simulink model "aero2_position_integral_R2021a"  (R2021a)
settings: Solver=ode1  StartTime=0.0  StopTime=60  FixedStep=0.002  RelTol=1e-3
model workspace (MAT data in the model file):
  Dpos = 5.83392170192
  Dq = 3.88928113461
  Kaw = 20
  Kff = 1
  Ki = 1.84164606325
  Kint = 7.35390515018
  Kp = 0.216370391856
  Kpos = 11.344880808
  Kq = 3.78162693601
  Kref = 3.78162693601
  ReferenceRate = [0 0.002 0.004 0.006 0.008 0.01 0.012 0.014 0.016 0.018 0.02 0.022 ... (90003 elements, 30001x3)]
  U_h : timeseries (value not decoded)
  U_v : timeseries (value not decoded)
  X0 = [0; 0; 0; 0]
  meas_on = 0
(part 2 of 2)

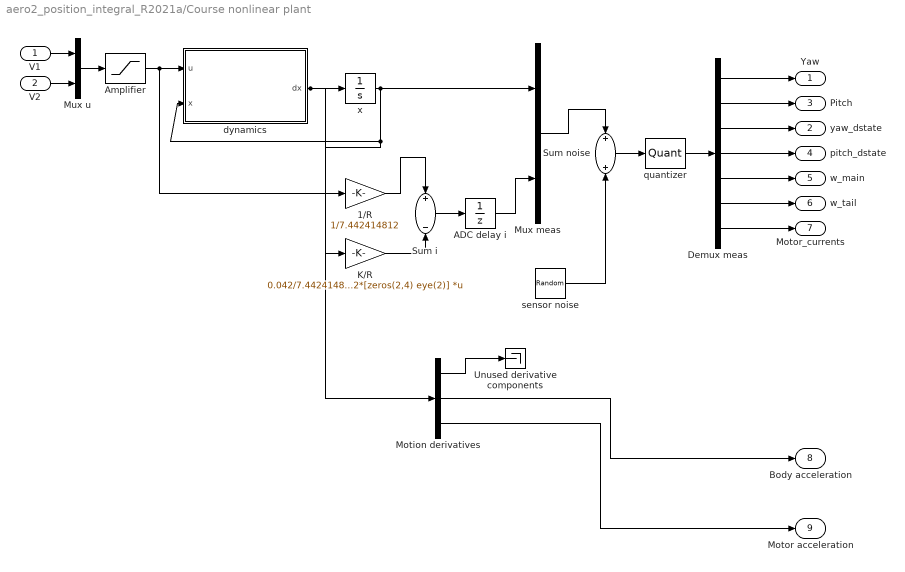
== system aero2_position_integral_R2021a/Course nonlinear plant ==
  V1 : Inport
  V2 : Inport  Port=2
  1/R : Gain  Gain=1/7.442414812
  ADC delay i : UnitDelay  InitialCondition=[0;0]  SampleTime=0.002
  Amplifier : Saturate  UpperLimit=24  LowerLimit=-24
  Demux meas : Demux  Outputs=[1 1 1 1 1 1 2]
  K/R : Gain  Gain=0.042/7.442414812*[zeros(2,4) eye(2)]  Multiplication=Matrix(K*u)
  Motion derivatives : Demux  Outputs=[2 2 2]
  Mux meas : Mux  Inputs=[6 2]
  Mux u : Mux  Inputs=2
  Sum i : Sum  Inputs=+-
  Sum noise : Sum
  Unused derivative components : Terminator
  dynamics : MATLAB Function  TreatAsAtomicUnit=on
  quantizer : Quantizer  QuantizationInterval=max((meas)*[0.0015339807878856412;0.0030679615757712823;0.001;0.001;0.050000000000000003;0.050000000000000003;0.001;0.001], 1e-12)
  sensor noise : RandomNumber  Mean=zeros(8,1)  Variance=((meas)*[0.0005;0.0005;0.005;0.005;0.3;0.3;0.01;0.01]).^2  Seed=[61027;18839;4421;30893;23341;7781;51117;9013]  SampleTime=0.002
  x : Integrator  InitialCondition=zeros(6,1)
  Yaw : Outport
  yaw_dstate : Outport  Port=2
  Pitch : Outport  Port=3
  pitch_dstate : Outport  Port=4
  w_main : Outport  Port=5
  w_tail : Outport  Port=6
  Motor_currents : Outport  Port=7
  Body acceleration : Outport  Port=8
  Motor acceleration : Outport  Port=9
  wires:
  Demux meas/7 -> Motor_currents/1
  Demux meas/6 -> w_tail/1
  Demux meas/5 -> w_main/1
  Demux meas/4 -> pitch_dstate/1
  Demux meas/2 -> Pitch/1
  Demux meas/3 -> yaw_dstate/1
  Demux meas/1 -> Yaw/1
  quantizer/1 -> Demux meas/1
  Sum noise/1 -> quantizer/1
  sensor noise/1 -> Sum noise/2
  Mux meas/1 -> Sum noise/1
  ADC delay i/1 -> Mux meas/2
  Sum i/1 -> ADC delay i/1
  K/R/1 -> Sum i/2
  1/R/1 -> Sum i/1
  x/1 -> K/R/1, dynamics/2(x), Mux meas/1
  dynamics/1(dx) -> x/1, Motion derivatives/1
  Amplifier/1 -> 1/R/1, dynamics/1(u)
  Mux u/1 -> Amplifier/1
  V2/1 -> Mux u/2
  V1/1 -> Mux u/1
  Motion derivatives/1 -> Unused derivative components/1
  Motion derivatives/2 -> Body acceleration/1
  Motion derivatives/3 -> Motor acceleration/1

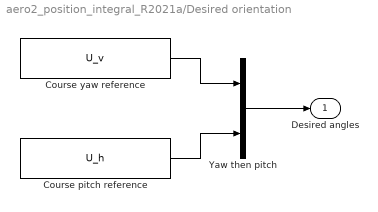
== system aero2_position_integral_R2021a/Desired orientation ==
  Course pitch reference : FromWorkspace  VariableName=U_h  OutputAfterFinalValue=Holding final value
  Course yaw reference : FromWorkspace  VariableName=U_v  OutputAfterFinalValue=Holding final value
  Yaw then pitch : Mux  Inputs=2
  Desired angles : Outport
  wires:
  Course yaw reference/1 -> Yaw then pitch/1
  Course pitch reference/1 -> Yaw then pitch/2
  Yaw then pitch/1 -> Desired angles/1

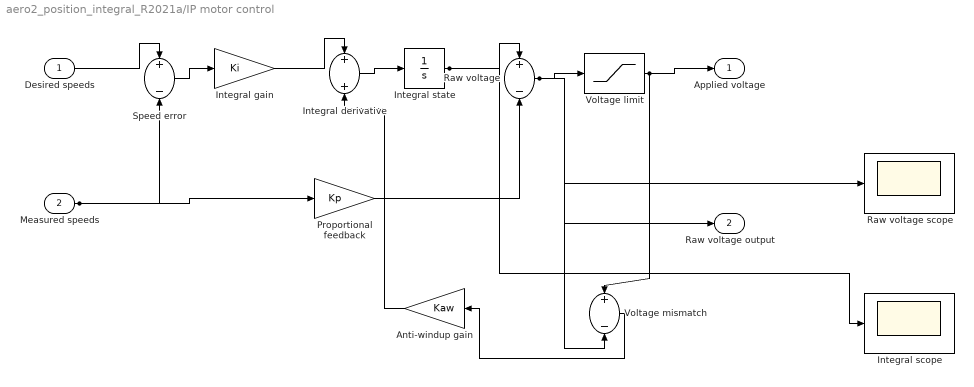
== system aero2_position_integral_R2021a/IP motor control ==
  Desired speeds : Inport
  Measured speeds : Inport  Port=2
  Anti-windup gain : Gain  Gain=Kaw
  Integral derivative : Sum
  Integral gain : Gain  Gain=Ki
  Integral scope : Scope
  Integral state : Integrator  InitialCondition=[0;0]
  Proportional feedback : Gain  Gain=Kp
  Raw voltage : Sum  Inputs=+-
  Raw voltage scope : Scope
  Speed error : Sum  Inputs=+-
  Voltage limit : Saturate  UpperLimit=24  LowerLimit=-24
  Voltage mismatch : Sum  Inputs=+-
  Applied voltage : Outport
  Raw voltage output : Outport  Port=2
  wires:
  Desired speeds/1 -> Speed error/1
  Measured speeds/1 -> Speed error/2, Proportional feedback/1
  Speed error/1 -> Integral gain/1
  Integral gain/1 -> Integral derivative/1
  Integral derivative/1 -> Integral state/1
  Integral state/1 -> Raw voltage/1, Integral scope/1
  Proportional feedback/1 -> Raw voltage/2
  Raw voltage/1 -> Voltage limit/1, Voltage mismatch/2, Raw voltage scope/1, Raw voltage output/1
  Voltage limit/1 -> Applied voltage/1, Voltage mismatch/1
  Voltage mismatch/1 -> Anti-windup gain/1
  Anti-windup gain/1 -> Integral derivative/2

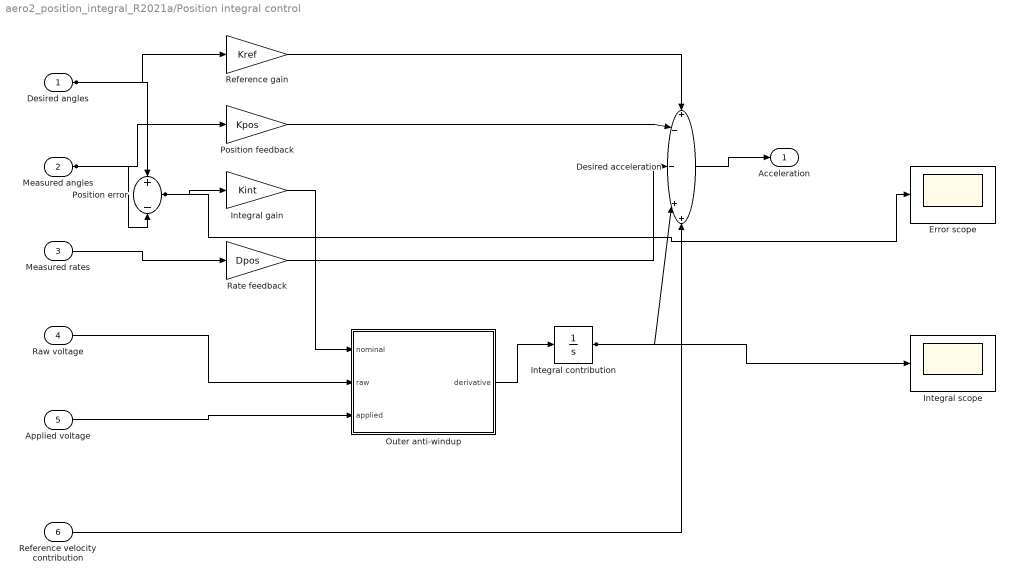
== system aero2_position_integral_R2021a/Position integral control ==
  Desired angles : Inport
  Measured angles : Inport  Port=2
  Measured rates : Inport  Port=3
  Raw voltage : Inport  Port=4
  Applied voltage : Inport  Port=5
  Reference velocity contribution : Inport  Port=6
  Desired acceleration : Sum  Inputs=+--++
  Error scope : Scope
  Integral contribution : Integrator  InitialCondition=[0;0]
  Integral gain : Gain  Gain=Kint
  Integral scope : Scope
  Outer anti-windup : MATLAB Function  TreatAsAtomicUnit=on
  Position error : Sum  Inputs=+-
  Position feedback : Gain  Gain=Kpos
  Rate feedback : Gain  Gain=Dpos
  Reference gain : Gain  Gain=Kref
  Acceleration : Outport
  wires:
  Desired angles/1 -> Position error/1, Reference gain/1
  Measured angles/1 -> Position error/2, Position feedback/1
  Measured rates/1 -> Rate feedback/1
  Position error/1 -> Integral gain/1, Error scope/1
  Integral gain/1 -> Outer anti-windup/1(nominal)
  Raw voltage/1 -> Outer anti-windup/2(raw)
  Applied voltage/1 -> Outer anti-windup/3(applied)
  Outer anti-windup/1(derivative) -> Integral contribution/1
  Reference gain/1 -> Desired acceleration/1
  Position feedback/1 -> Desired acceleration/2
  Rate feedback/1 -> Desired acceleration/3
  Integral contribution/1 -> Desired acceleration/4, Integral scope/1
  Desired acceleration/1 -> Acceleration/1
  Reference velocity contribution/1 -> Desired acceleration/5

== matlab function aero2_position_integral_R2021a/Course nonlinear plant/dynamics ==
  data: u input; dx output; x input
function dx = fcn(u, x)
%% Simplified twin-rotor model of aero2_model.pdf (2-DOF body + first-order motors)
p = struct('Jph', 0.64070000000000005, ...
    'jph', 0.01, ...
    'Jth', 0.71640000000000004, ...
    'G', 0.025399999999999999, ...
    'kT', 4.2486999999999997e-06, ...
    'kF', 2.5525999999999999e-05, ...
    'L', 0.16700000000000001, ...
    'Cor', 0.63070000000000004, ...
    'Dph', 0, ...
    'Dth', 0, ...
    'aw', 5.7800000000000002, ...
    'bw', 96.531999999999996);
dx = tr_simp_dyn(x, u, p);
end

function dx = tr_simp_dyn(x, u, p)
%TR_SIMP_DYN  Simplified twin-rotor model with voltage inputs (aero2_model.pdf).
%   Body: reduced 2-DOF model, eq. (simp)
%     Mq(th) [ddpsi; ddth] + cq + Bq dq + gq = Gamma(th) [wm|wm|; wt|wt|]
%   with cq = [-Cor sin(2th) dth dpsi; 1/2 Cor sin(2th) dpsi^2]
%   (no gyroscopic coupling, no motor reaction channel, s_m=+1, s_t=-1).
%   Rotors: first-order motor model of the hand-out
%     dw = -aw w + bw v
%   State x = [psi, theta, dpsi, dtheta, wm, wt], input u = [Um, Ut].
%   p: Jph jph Jth Dph Dth Cor L G kF kT aw bw (psim of tr_instructor_params).

    th = x(2);  dps = x(3);  dth = x(4);
    c = cos(th);  s = sin(th);
    tau = [x(5)*abs(x(5)); x(6)*abs(x(6))];

    Ms  = [p.Jph*c^2 + p.jph*s^2, 0; 0, p.Jth];
    Cs  = [-p.Cor*sin(2*th)*dth*dps; 0.5*p.Cor*sin(2*th)*dps^2];
    Ds  = [p.Dph*dps; p.Dth*dth];
    Gs  = [0; p.G*s];
    Gam = [c 0; 0 1]*[-p.kT, p.L*p.kF; p.L*p.kF, p.kT];
    ddq = Ms\(Gam*tau - Cs - Ds - Gs);

    dw  = -p.aw*x(5:6) + p.bw*u(:);
    dx  = [x(3:4); ddq; dw];
end

== matlab function aero2_position_integral_R2021a/Mechanical inverse ==
  data: q input; omegaDesired output; dq input; a input
function omegaDesired = aero2_feedback_linearization(q, dq, a)
%AERO2_FEEDBACK_LINEARIZATION Ideal motor tracking: choose omega for q_ddot=a.
% The signed square root is defined at zero but has no finite derivative there.
p = aero2_mechanical_parameters;
assert(abs(q(2)) <= p.pitchLimit, 'Pitch envelope exceeded (limit 60 deg).');
[M, c, g, Gamma] = aero2_mechanical_terms(q, dq);
s = Gamma\(M*a+c+g);
omegaDesired = sign(s).*sqrt(abs(s));
end

function [M, c, g, Gamma] = aero2_mechanical_terms(q, dq)
%AERO2_MECHANICAL_TERMS M*q_ddot+c+g=Gamma*(omega.*abs(omega)).
% Signal order: q=[yaw;pitch], dq=[yaw rate;pitch rate], omega=[main;tail].
p = aero2_mechanical_parameters;
theta = q(2);
cor = p.Jyaw-p.jyaw;
M = [p.Jyaw*cos(theta)^2+p.jyaw*sin(theta)^2, 0; 0, p.Jpitch];
c = [-cor*sin(2*theta)*dq(2)*dq(1); ...
    0.5*cor*sin(2*theta)*dq(1)^2];
g = [0; p.gravity*sin(theta)];
Gamma = [cos(theta), 0; 0, 1]*[-p.kt, p.lever*p.kf; p.lever*p.kf, p.kt];
end

function p = aero2_mechanical_parameters
%AERO2_MECHANICAL_PARAMETERS Simplified course model, Part II, pages 4-5.
p.Jyaw = 0.6407;
p.jyaw = 0.01;
p.Jpitch = 0.7164;
p.gravity = 0.0254;
p.kt = 4.2487e-6;
p.kf = 2.5526e-5;
p.lever = 0.167;
p.pitchLimit = pi/3; % Simulation envelope, not an approved hardware limit.
p.initialState = [0.1; 0.2; -0.05; 0.04]; % [yaw; pitch; yaw rate; pitch rate].
p.acceleration = [0.15; -0.1];
p.step = 0.002;
end

== matlab function aero2_position_integral_R2021a/Position integral control/Outer anti-windup ==
  data: nominal input; derivative output; raw input; applied input
function derivative = outer_aw(nominal,raw,applied)
derivative=nominal;
if any(abs(raw-applied)>1e-8)
    derivative=zeros(2,1);
end
end
